simulink model "cartPendulum"  (R2026a)
settings: Solver=ode45  StopTime=50  RelTol=1e-5
values from neighbouring files (symbols this model uses):
  g = 9.81    [cartPendulum_param.m]
  l = 0.5    [cartPendulum_param.m]
  m = 0.5    [cartPendulum_param.m]
  M = 1    [cartPendulum_param.m]
settings Model: Creator=admin  LastModifiedBy=juraj

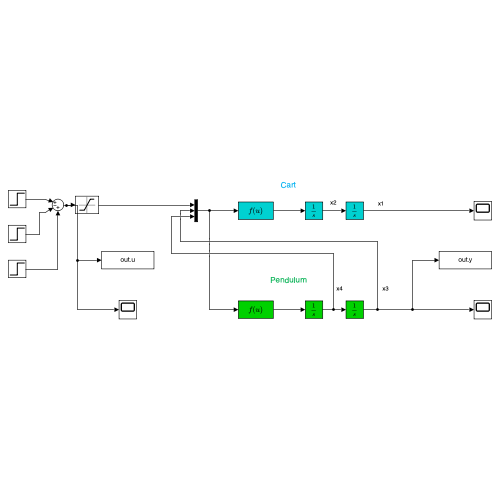
[thumbnail: Simulink's stored preview of the top-level diagram]
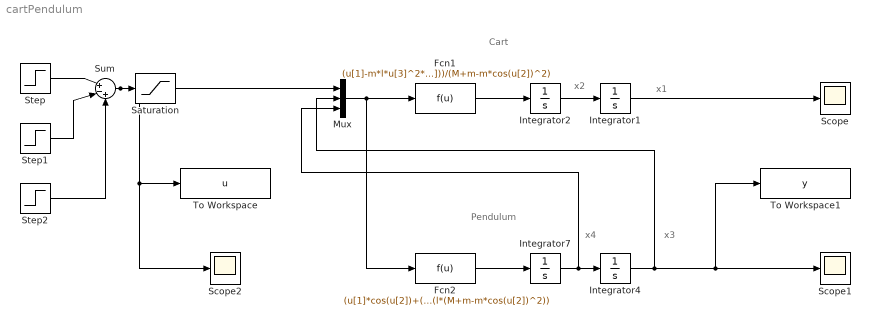
== system cartPendulum ==
  note: x3
  note: x4
  note: Cart
  note: x1
  note: x2
  note: Pendulum
  Fcn1 : Fcn  Expr=(u[1]-m*l*u[3]^2*sin(u[2])+m*g*sin(u[2])*cos(u[2]))/(M+m-m*cos(u[2])^2)
  Fcn2 : Fcn  Expr=(u[1]*cos(u[2])+(M+m)*g*sin(u[2])-m*l*u[3]^2*sin(u[2])*cos(u[2]))/(l*(M+m-m*cos(u[2])^2))
  Integrator{1..2,4,7} (4 alike) : Integrator
  Mux : Mux  Inputs=3
  Saturation : Saturate  UpperLimit=20  LowerLimit=-20
  Scope : Scope
      settings: ActiveDisplayYMinimum=-0.39789166018100353  ActiveDisplayYMaximum=1.9886253034069823
  Scope1 : Scope
      settings: ActiveDisplayYMinimum=-58.1162949716433  ActiveDisplayYMaximum=20.417659592824528
  Scope2 : Scope
      settings: ActiveDisplayYMinimum=-0.012499999999999999  ActiveDisplayYMaximum=0.012499999999999999  DataLoggingVariableName=ScopeData2
  Step : Step  Time=10  InitialValue=5e-3  FinalValue=1e-2  SampleTime=.1
  Step1 : Step  Time=20  FinalValue=2e-2  SampleTime=0.1
  Step2 : Step  Time=40  FinalValue=5e-3  SampleTime=0.1
  Sum : Sum  Inputs=|+-+
  To Workspace : ToWorkspace  VariableName=u  SaveFormat=Timeseries  SampleTime=-1
  To Workspace1 : ToWorkspace  VariableName=y  SaveFormat=Timeseries  SampleTime=-1
  wires:
  Integrator7/1 -> Mux/3, Integrator4/1
  Sum/1 -> Scope2/1, To Workspace/1, Saturation/1
  Integrator2/1 -> Integrator1/1
  Mux/1 -> Fcn2/1, Fcn1/1
  Fcn1/1 -> Integrator2/1
  Integrator4/1 -> To Workspace1/1, Scope1/1, Mux/2
  Fcn2/1 -> Integrator7/1
  Integrator1/1 -> Scope/1
  Step/1 -> Sum/1
  Step1/1 -> Sum/2
  Step2/1 -> Sum/3
  Saturation/1 -> Mux/1
